simulink model "fw_adc_scaling"  (R2026b)
settings: Solver=VariableStepAuto
undefined symbols (not defined in the file or in its folder): P, Ts
settings Model: Creator=aomar  LastModifiedBy=aomar

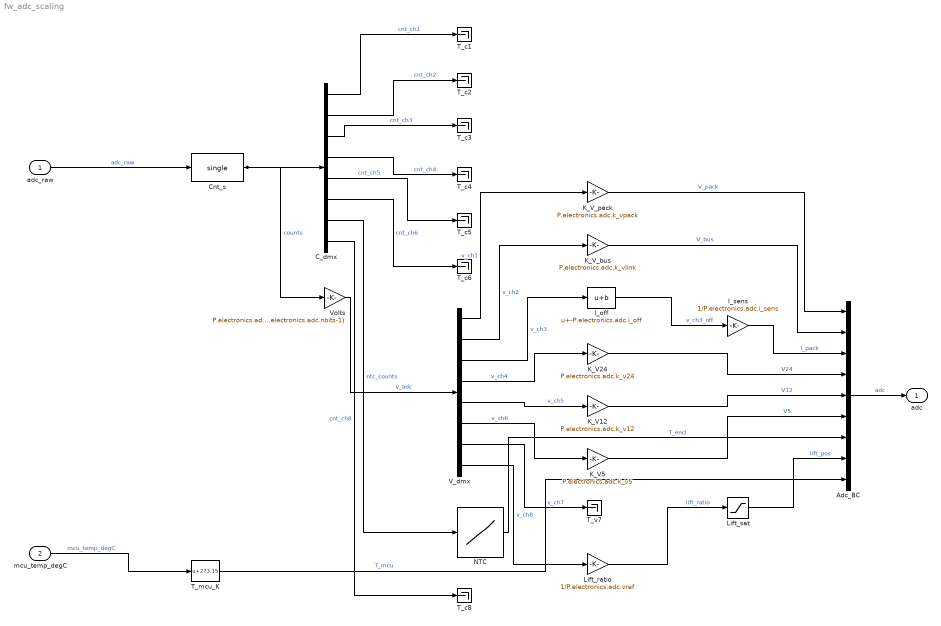
== system fw_adc_scaling ==
  adc_raw : Inport  OutDataTypeStr=uint16  PortDimensions=8  SampleTime=Ts.comm
  mcu_temp_degC : Inport  Port=2  OutDataTypeStr=single  SampleTime=Ts.comm
  Adc_BC : BusCreator  Inputs=9
  C_dmx : Demux  Outputs=8
  Cnt_s : DataTypeConversion  OutDataTypeStr=single  RndMeth=Round
  I_off : Bias  Bias=-P.electronics.adc.i_off  SaturateOnIntegerOverflow=off
  I_sens : Gain  Gain=1/P.electronics.adc.i_sens
  K_V12 : Gain  Gain=P.electronics.adc.k_v12
  K_V24 : Gain  Gain=P.electronics.adc.k_v24
  K_V5 : Gain  Gain=P.electronics.adc.k_v5
  K_V_bus : Gain  Gain=P.electronics.adc.k_vlink
  K_V_pack : Gain  Gain=P.electronics.adc.k_vpack
  Lift_ratio : Gain  Gain=1/P.electronics.adc.vref
  Lift_sat : Saturate  UpperLimit=1  LowerLimit=0
  NTC : Lookup_n-D  NumberOfTableDimensions=1  BreakpointsForDimension1=P.electronics.adc.ntc_lut_counts  Table=P.electronics.adc.ntc_lut_K  ExtrapMethod=Clip  InternalRulePriority=Speed  OutDataTypeStr=single  RndMeth=Simplest
  T_c{1..6,8} (7 alike) : Terminator
  T_mcu_K : Bias  Bias=273.15  SaturateOnIntegerOverflow=off
  T_v7 : Terminator
  V_dmx : Demux  Outputs=8
  Volts : Gain  Gain=P.electronics.adc.vref/(2^P.electronics.adc.nbits-1)
  adc : Outport
  wires:
  adc_raw/1 -> Cnt_s/1  "adc_raw"
  mcu_temp_degC/1 -> T_mcu_K/1  "mcu_temp_degC"
  T_mcu_K/1 -> Adc_BC/9  "T_mcu"
  Cnt_s/1 -> Volts/1, C_dmx/1  "counts"
  C_dmx/1 -> T_c1/1  "cnt_ch1"
  C_dmx/2 -> T_c2/1  "cnt_ch2"
  C_dmx/3 -> T_c3/1  "cnt_ch3"
  C_dmx/4 -> T_c4/1  "cnt_ch4"
  C_dmx/5 -> T_c5/1  "cnt_ch5"
  C_dmx/6 -> T_c6/1  "cnt_ch6"
  C_dmx/7 -> NTC/1  "ntc_counts"
  C_dmx/8 -> T_c8/1  "cnt_ch8"
  Volts/1 -> V_dmx/1  "v_adc"
  V_dmx/1 -> K_V_pack/1  "v_ch1"
  V_dmx/2 -> K_V_bus/1  "v_ch2"
  V_dmx/3 -> I_off/1  "v_ch3"
  V_dmx/4 -> K_V24/1  "v_ch4"
  V_dmx/5 -> K_V12/1  "v_ch5"
  V_dmx/6 -> K_V5/1  "v_ch6"
  V_dmx/7 -> T_v7/1  "v_ch7"
  V_dmx/8 -> Lift_ratio/1  "v_ch8"
  NTC/1 -> Adc_BC/7  "T_encl"
  K_V_pack/1 -> Adc_BC/1  "V_pack"
  K_V_bus/1 -> Adc_BC/2  "V_bus"
  K_V24/1 -> Adc_BC/4  "V24"
  K_V12/1 -> Adc_BC/5  "V12"
  K_V5/1 -> Adc_BC/6  "V5"
  Lift_ratio/1 -> Lift_sat/1  "lift_ratio"
  I_off/1 -> I_sens/1  "v_ch3_off"
  I_sens/1 -> Adc_BC/3  "I_pack"
  Lift_sat/1 -> Adc_BC/8  "lift_pos"
  Adc_BC/1 -> adc/1  "adc"
